simulink model "POWERTRAIN"  (R2026a)
settings: Solver=VariableStepAuto  StopTime=120
InitFcn:
  | Initialize_Project;
undefined symbols (not defined in the file): EV
libraries: SignalEditorBlockLib x1, slpidlib x1
settings Model: Creator=surya  LastModifiedBy=surya

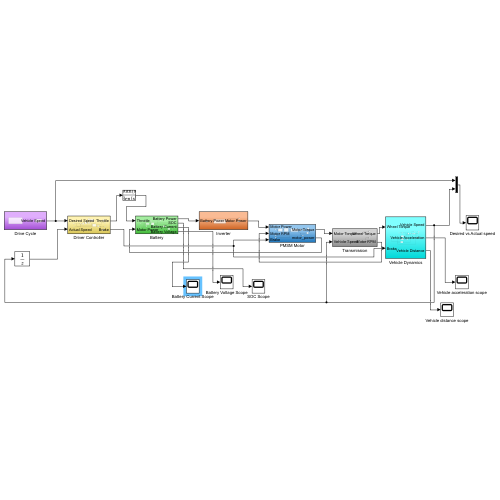
[thumbnail: Simulink's stored preview of the top-level diagram]
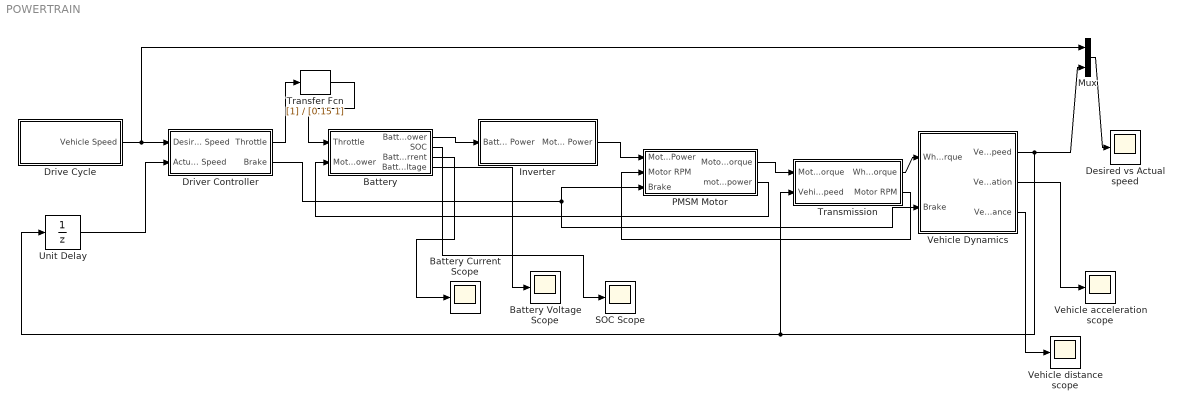
== system POWERTRAIN ==
  Battery : Subsystem
  Battery Current Scope : Scope
      settings: ActiveDisplayYMinimum=-12.119623125546823  ActiveDisplayYMaximum=33.082292003345252  DataLoggingVariableName=ScopeData17
  Battery Voltage Scope : Scope
      settings: ActiveDisplayYMinimum=399.7977387135885  ActiveDisplayYMaximum=400.022473476268  DataLoggingVariableName=ScopeData11
  Desired vs Actual speed : Scope
      settings: ActiveDisplayYMinimum=-2.532730452502121  ActiveDisplayYMaximum=22.794574072519094
  Drive Cycle : Subsystem
  Driver Controller : Subsystem
  Inverter : Subsystem
  Mux : Mux  Inputs=2
  PMSM Motor : Subsystem
  SOC Scope : Scope
      settings: ActiveDisplayYMinimum=99.747173391985541  ActiveDisplayYMaximum=100.02809184533494
  Transfer Fcn : TransferFcn  Denominator=[0.15 1]
  Transmission : Subsystem
  Unit Delay : UnitDelay  SampleTime=-1
  Vehicle Dynamics : Subsystem
  Vehicle acceleration scope : Scope
      settings: ActiveDisplayYMinimum=-1.1905303240766103  ActiveDisplayYMaximum=1.7943093242123052  DataLoggingVariableName=ScopeData6
  Vehicle distance scope : Scope
      settings: ActiveDisplayYMinimum=-118.29137386717078  ActiveDisplayYMaximum=1064.6223648045373  DataLoggingVariableName=ScopeData7
  wires:
  Drive Cycle/1(Vehicle Speed) -> Mux/1, Driver Controller/1(Desired Speed)
  Unit Delay/1 -> Driver Controller/2(Actual Speed)
  Driver Controller/1(Throttle) -> Transfer Fcn/1
  Battery/1(Battery Power) -> Inverter/1(Battery Power)
  Inverter/1(Motor Power) -> PMSM Motor/1(Motor Power)
  PMSM Motor/1(Motor Torque) -> Transmission/1(Motor Torque)
  Transmission/1(Wheel Torque) -> Vehicle Dynamics/1(Wheel Torque)
  Vehicle Dynamics/1(Vehicle Speed) -> Transmission/2(Vehicle Speed), Unit Delay/1, Mux/2
  Battery/2(SOC) -> SOC Scope/1
  Vehicle Dynamics/2(Vehicle Acceleration) -> Vehicle acceleration scope/1
  Vehicle Dynamics/3(Vehicle Distance) -> Vehicle distance scope/1
  Transmission/2(Motor RPM) -> PMSM Motor/2(Motor RPM)
  Transfer Fcn/1 -> Battery/1(Throttle)
  Driver Controller/2(Brake) -> PMSM Motor/3(Brake), Vehicle Dynamics/2(Brake)
  PMSM Motor/2(motor_power) -> Battery/2(Motor Power)
  Battery/3(Battery Current) -> Battery Current Scope/1
  Mux/1 -> Desired vs Actual speed/1
  Battery/4(Battery Voltage) -> Battery Voltage Scope/1

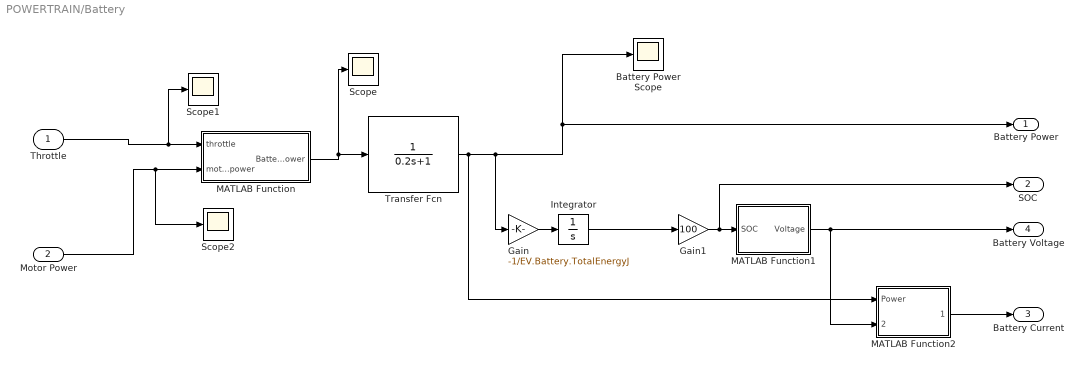
== system POWERTRAIN/Battery ==
  Throttle : Inport
  Motor Power : Inport  Port=2
  Battery Power Scope : Scope
      settings: ActiveDisplayYMinimum=-1  ActiveDisplayYMaximum=1  DataLoggingVariableName=ScopeData2
  Gain : Gain  Gain=-1/EV.Battery.TotalEnergyJ
  Gain1 : Gain  Gain=100
  Integrator : Integrator  InitialCondition=EV.Battery.InitialSOC/100  LimitOutput=on  UpperSaturationLimit=1  LowerSaturationLimit=0
  MATLAB Function : MATLAB Function  TreatAsAtomicUnit=on
  MATLAB Function1 : MATLAB Function  TreatAsAtomicUnit=on
  MATLAB Function2 : MATLAB Function  TreatAsAtomicUnit=on
  Scope : Scope
      settings: ActiveDisplayYMinimum=-1  ActiveDisplayYMaximum=1  DataLoggingVariableName=ScopeData13
  Scope1 : Scope
      settings: ActiveDisplayYMinimum=-1  ActiveDisplayYMaximum=1  DataLoggingVariableName=ScopeData2
  Scope2 : Scope
      settings: ActiveDisplayYMinimum=-1  ActiveDisplayYMaximum=1  DataLoggingVariableName=ScopeData3
  Transfer Fcn : TransferFcn  Denominator=[0.2 1]
  Battery Power : Outport
  SOC : Outport  Port=2
  Battery Current : Outport  Port=3
  Battery Voltage : Outport  Port=4
  wires:
  Throttle/1 -> Scope1/1, MATLAB Function/1(throttle)
  MATLAB Function/1(BatteryPower) -> Scope/1, Transfer Fcn/1
  Transfer Fcn/1 -> MATLAB Function2/1(Power), Gain/1, Battery Power Scope/1, Battery Power/1
  Gain/1 -> Integrator/1
  Integrator/1 -> Gain1/1
  Gain1/1 -> SOC/1, MATLAB Function1/1(SOC)
  Motor Power/1 -> Scope2/1, MATLAB Function/2(motor_power)
  MATLAB Function1/1(Voltage) -> Battery Voltage/1, MATLAB Function2/2(Voltage)
  MATLAB Function2/1(Current) -> Battery Current/1

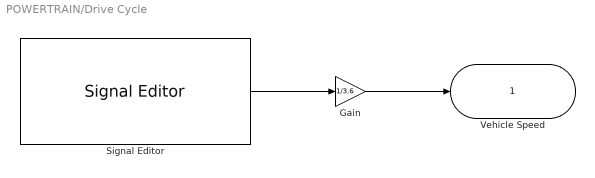
== system POWERTRAIN/Drive Cycle ==
  Gain : Gain  Gain=1/3.6
  Signal Editor : SignalEditorBlockLib/Signal Editor  FileName=C:\Users\surya\OneDrive\Documents\Smart-EV-Powertrain-Simulator\DriveCycles\DriveCycle.mat  ActiveScenario=Scenario  ActiveSignal=Vehicle Speed  IsBus=off  OutputBusObjectStr=Bus: BusObject  SampleTime=0  ZeroCross=off  OutputAfterFinalValue=Setting to zero  Unit=inherit  PreserveSignalName=on  ApplySigPropsToAllScenarios=on  ApplySigPropsToAllSignals=off  SignalPropertySource=Dialog parameters
  Vehicle Speed : Outport
  wires:
  Signal Editor/1 -> Gain/1
  Gain/1 -> Vehicle Speed/1

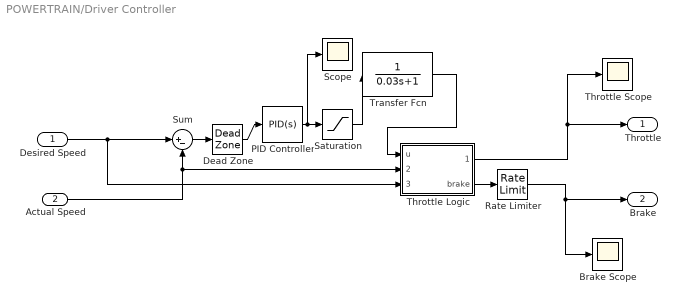
== system POWERTRAIN/Driver Controller ==
  Desired Speed : Inport
  Actual Speed : Inport  Port=2
  Brake Scope : Scope
      settings: ActiveDisplayYMinimum=-1  ActiveDisplayYMaximum=1  DataLoggingVariableName=ScopeData12
  Dead Zone : DeadZone  LowerValue=-0.1  UpperValue=0.1
  PID Controller : slpidlib/PID Controller  Controller=PID  Form=Parallel  TimeDomain=Continuous-time  UseExternalTs=off  SampleTime=-1  IntegratorMethod=Forward Euler  FilterMethod=Forward Euler  ControllerParametersSource=internal  P=0.03  I=0.001  UseKiTs=off  D=0.001  UseExternalDerivativeSource=off  N=20  UseFilter=on  TunerSelectOption=Transfer Function Based (PID Tuner App)  InitialConditionSource=internal  InitialConditionForIntegrator=0  InitialConditionForFilter=0  DifferentiatorICPrevScaledInput=0  ExternalReset=none  TrackingMode=off  Kt=1  LimitOutput=on  SatLimitsSource=internal  UpperSaturationLimit=1  LowerSaturationLimit=-1  LinearizeAsGain=on  AntiWindupMode=back-calculation  Kb=1  LimitIntegrator=off  UpperIntegratorSaturationLimit=inf  LowerIntegratorSaturationLimit=-inf  POutMin=[]  POutMax=[]  IOutMin=[]  IOutMax=[]  DOutMin=[]  DOutMax=[]  NOutMin=[]  NOutMax=[]  SumOutMin=[]  SumOutMax=[]  SaturationOutMin=[]  SaturationOutMax=[]  PParamMin=[]  PParamMax=[]  IParamMin=[]  IParamMax=[]  DParamMin=[]  DParamMax=[]  NParamMin=[]  NParamMax=[]  KbParamMin=[]  KbParamMax=[]  KtParamMin=[]  KtParamMax=[]  KbOutMin=[]  KbOutMax=[]  KtOutMin=[]  KtOutMax=[]  IntegratorOutMin=[]  IntegratorOutMax=[]  FilterOutMin=[]  FilterOutMax=[]  SumI1OutMin=[]  SumI1OutMax=[]  SumI2OutMin=[]  SumI2OutMax=[]  SumI3OutMin=[]  SumI3OutMax=[]  SumI4OutMin=[]  SumI4OutMax=[]  SumDOutMin=[]  SumDOutMax=[]  DifferentiatorOutMin=[]  DifferentiatorOutMax=[]  FilterDiffOutCoefMin=[]  FilterDiffOutCoefMax=[]  ReciprocalOutMin=[]  ReciprocalOutMax=[]  SumDenOutMin=[]  SumDenOutMax=[]  SumNumOutMin=[]  SumNumOutMax=[]  DivideOutMin=[]  DivideOutMax=[]  UdiffTsProdOutMin=[]  UdiffTsProdOutMax=[]  NTsProdOutMin=[]  NTsProdOutMax=[]  UintegralTsProdOutMin=[]  UintegralTsProdOutMax=[]  UngainTsProdOutMin=[]  UngainTsProdOutMax=[]  ClampingZeroOutDataTypeStr=Inherit: Inherit via back propagation  ClampingZeroOutMin=[]  ClampingZeroOutMax=[]  FilterDenConstantOutDataTypeStr=Inherit: Inherit via back propagation  FilterDenConstantOutMin=[]  FilterDenConstantOutMax=[]  PCopyOutDataTypeStr=Inherit: Inherit via back propagation  PCopyOutMin=[]  PCopyOutMax=[]  NCopyOutDataTypeStr=Inherit: Inherit via back propagation  NCopyOutMin=[]  NCopyOutMax=[]  IntegratorContinuousStateAttributes=''  IntegratorStateMustResolveToSignalObject=off  IntegratorRTWStateStorageClass=Auto  FilterContinuousStateAttributes=''  FilterStateMustResolveToSignalObject=off  FilterRTWStateStorageClass=Auto  ParallelPVariant=InternalParameters  IdealPVariant=Disabled  IVariant=InternalParameters  DVariant=InternalParameters  IntegratorVariant=Continuous  SatVariant=Enabled  AWVariant=BackCalculation  PCopyVariant=Disabled  TRVariant=Disabled  FdbkBlocksVariant=Forward  IdealPFdbkVariant=Disabled  SatFdbkVariant=Disabled  DerivativeFilterVariant=ContFilter  NVariant=InternalParameters  NCopyVariant=Disabled  FilterICVariant=InternalICsFilter  IntegratorICVariant=InternalICs  ExternalResetVariant=Disabled  TRSumVariant=Passthrough  SumFdbkVariant=Disabled  SumVariant=Sum_PID  TsampFilterVariant=InternalTs  TsampNgainVariant=Passthrough  TsampIntegralVariant=Disabled_SignalSpec  ExternalSaturationOutDataTypeStr=Inherit: Same as second input  DerivativeSourceVariant=ErrorSignal  PreIntVariant=InternalPreInt
  Rate Limiter : RateLimiter  RisingSlewLimit=0.05  FallingSlewLimit=-0.05  SampleTimeMode=inherited
  Saturation : Saturate  UpperLimit=1  LowerLimit=-1
  Scope : Scope
      settings: ActiveDisplayYMinimum=-1  ActiveDisplayYMaximum=1  DataLoggingVariableName=ScopeData4
  Sum : Sum  Inputs=|+-
  Throttle Logic : MATLAB Function  TreatAsAtomicUnit=on
  Throttle Scope : Scope
      settings: ActiveDisplayYMinimum=-0.028171879428741577  ActiveDisplayYMaximum=0.25354691485867425  DataLoggingVariableName=ScopeData10
  Transfer Fcn : TransferFcn  Denominator=[0.03 1]
  Throttle : Outport  VectorParamsAs1DForOutWhenUnconnected=off
  Brake : Outport  Port=2
  wires:
  Desired Speed/1 -> Throttle Logic/3(desired_speed), Sum/1
  Sum/1 -> Dead Zone/1
  Throttle Logic/1(throttle) -> Throttle/1, Throttle Scope/1
  Actual Speed/1 -> Throttle Logic/2(actual_speed), Sum/2
  Dead Zone/1 -> PID Controller/1
  Throttle Logic/2(brake) -> Rate Limiter/1
  Rate Limiter/1 -> Brake Scope/1, Brake/1
  PID Controller/1 -> Scope/1, Saturation/1
  Saturation/1 -> Transfer Fcn/1
  Transfer Fcn/1 -> Throttle Logic/1(u)

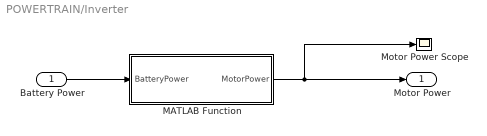
== system POWERTRAIN/Inverter ==
  Battery Power : Inport
  MATLAB Function : MATLAB Function  TreatAsAtomicUnit=on
  Motor Power Scope : Scope
      settings: ActiveDisplayYMinimum=-1  ActiveDisplayYMaximum=1  DataLoggingVariableName=ScopeData9
  Motor Power : Outport
  wires:
  Battery Power/1 -> MATLAB Function/1(BatteryPower)
  MATLAB Function/1(MotorPower) -> Motor Power Scope/1, Motor Power/1

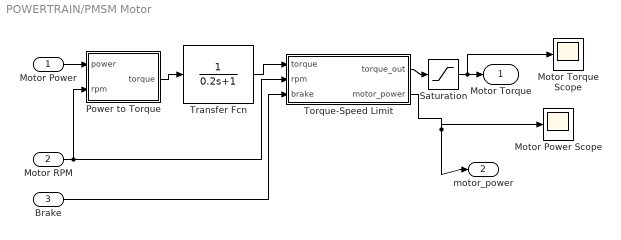
== system POWERTRAIN/PMSM Motor ==
  Motor Power : Inport
  Motor RPM : Inport  Port=2
  Brake : Inport  Port=3
  Motor Power Scope : Scope
      settings: ActiveDisplayYMinimum=-1  ActiveDisplayYMaximum=1  DataLoggingVariableName=ScopeData16
  Motor Torque Scope : Scope
      settings: ActiveDisplayYMinimum=-1  ActiveDisplayYMaximum=1  DataLoggingVariableName=ScopeData4
  Power to Torque : MATLAB Function  TreatAsAtomicUnit=on
  Saturation : Saturate  UpperLimit=EV.Motor.PeakTorque  LowerLimit=-EV.Motor.PeakTorque
  Torque-Speed Limit : MATLAB Function  TreatAsAtomicUnit=on
  Transfer Fcn : TransferFcn  Denominator=[0.2 1]
  Motor Torque : Outport
  motor_power : Outport  Port=2
  wires:
  Motor Power/1 -> Power to Torque/1(power)
  Power to Torque/1(torque) -> Transfer Fcn/1
  Transfer Fcn/1 -> Torque-Speed Limit/1(torque)
  Saturation/1 -> Motor Torque Scope/1, Motor Torque/1
  Torque-Speed Limit/1(torque_out) -> Saturation/1
  Motor RPM/1 -> Power to Torque/2(rpm), Torque-Speed Limit/2(rpm)
  Brake/1 -> Torque-Speed Limit/3(brake)
  Torque-Speed Limit/2(motor_power) -> motor_power/1, Motor Power Scope/1

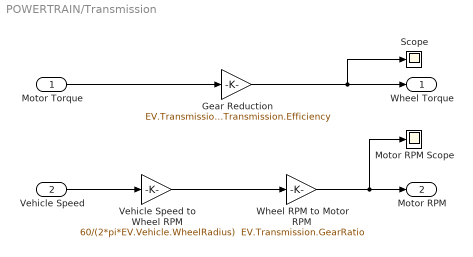
== system POWERTRAIN/Transmission ==
  Motor Torque : Inport
  Vehicle Speed : Inport  Port=2
  Gear Reduction : Gain  Gain=EV.Transmission.GearRatio * EV.Transmission.Efficiency
  Motor RPM Scope : Scope
      settings: ActiveDisplayYMinimum=-1  ActiveDisplayYMaximum=1  DataLoggingVariableName=ScopeData8
  Scope : Scope
      settings: ActiveDisplayYMinimum=-1  ActiveDisplayYMaximum=1  DataLoggingVariableName=ScopeData5
  Vehicle Speed to Wheel RPM : Gain  Gain=60/(2*pi*EV.Vehicle.WheelRadius)
  Wheel RPM to Motor RPM : Gain  Gain=EV.Transmission.GearRatio
  Wheel Torque : Outport
  Motor RPM : Outport  Port=2
  wires:
  Motor Torque/1 -> Gear Reduction/1
  Gear Reduction/1 -> Wheel Torque/1, Scope/1
  Vehicle Speed/1 -> Vehicle Speed to Wheel RPM/1
  Vehicle Speed to Wheel RPM/1 -> Wheel RPM to Motor RPM/1
  Wheel RPM to Motor RPM/1 -> Motor RPM Scope/1, Motor RPM/1

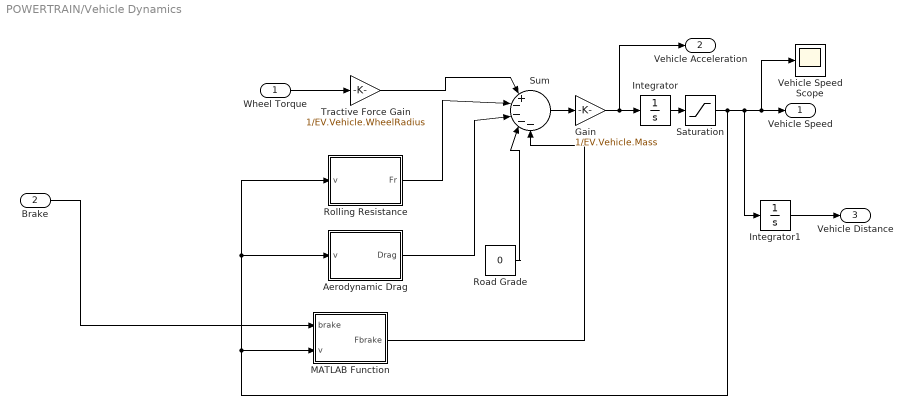
== system POWERTRAIN/Vehicle Dynamics ==
  Wheel Torque : Inport
  Brake : Inport  Port=2
  Aerodynamic Drag : MATLAB Function  TreatAsAtomicUnit=on
  Gain : Gain  Gain=1/EV.Vehicle.Mass
  Integrator : Integrator
  Integrator1 : Integrator
  MATLAB Function : MATLAB Function  TreatAsAtomicUnit=on
  Road Grade : Constant  Value=0
  Rolling Resistance : MATLAB Function  TreatAsAtomicUnit=on
  Saturation : Saturate  UpperLimit=EV.Requirements.TopSpeed  LowerLimit=0
  Sum : Sum  Inputs=|+----
  Tractive Force Gain : Gain  Gain=1/EV.Vehicle.WheelRadius
  Vehicle Speed Scope : Scope
      settings: ActiveDisplayYMinimum=-1  ActiveDisplayYMaximum=1  DataLoggingVariableName=ScopeData3
  Vehicle Speed : Outport
  Vehicle Acceleration : Outport  Port=2
  Vehicle Distance : Outport  Port=3
  wires:
  Wheel Torque/1 -> Tractive Force Gain/1
  Tractive Force Gain/1 -> Sum/1
  Rolling Resistance/1(Fr) -> Sum/2
  Sum/1 -> Gain/1
  Gain/1 -> Integrator/1, Vehicle Acceleration/1
  Integrator/1 -> Saturation/1
  Aerodynamic Drag/1(Drag) -> Sum/3
  Saturation/1 -> Integrator1/1, Vehicle Speed Scope/1, Vehicle Speed/1, Aerodynamic Drag/1(v), Rolling Resistance/1(v), MATLAB Function/2(v)
  Road Grade/1 -> Sum/4
  Integrator1/1 -> Vehicle Distance/1
  Brake/1 -> MATLAB Function/1(brake)
  MATLAB Function/1(Fbrake) -> Sum/5

== matlab function POWERTRAIN/Driver Controller/Throttle Logic ==
  data: u input; throttle output; brake output; actual_speed input; desired_speed input
function [throttle, brake] = fcn(u, actual_speed, desired_speed)

neutral = 0.02;      % Neutral zone around zero

throttle = 0.03;
brake = 0;

% Vehicle stopped
if desired_speed < 0.1 && actual_speed < 0.1

    throttle = 0;
    brake = 0;

    % Accelerate
elseif u > neutral

    throttle = min(u,1);
    brake = 0;

    % Brake
elseif u < -neutral

    throttle = 0;
    brake = min(-u,1);

    % Neutral (no throttle, no brake)
else

    throttle = 0;
    brake = 0;

end

== matlab function POWERTRAIN/PMSM Motor/Power to Torque ==
  data: power input; torque output; rpm input
function torque = fcn(power, rpm)

% Prevent division by zero
rpm_safe = max(abs(rpm),100);

% Convert RPM to rad/s
omega = rpm_safe * 2*pi/60;

% Calculate torque
torque = power / omega;

end

== matlab function POWERTRAIN/Battery/MATLAB Function ==
  data: throttle input; BatteryPower output; motor_power input
function BatteryPower = fcn(throttle,motor_power)

MaxPower = 50000;      % W
DischargeEff = 0.96;
ChargeEff = 0.90;

if motor_power < 0

    % Regenerative charging
    BatteryPower = motor_power * ChargeEff;

else

    RequestedPower = throttle * MaxPower;

    BatteryPower = RequestedPower / DischargeEff;

end

== matlab function POWERTRAIN/Vehicle Dynamics/Aerodynamic Drag ==
  data: v input; Drag output
function Drag = fcn(v)

rho = 1.225;
Cd  = 0.30;
A   = 2.40;

Drag = 0.5 * rho * Cd * A * v * abs(v);

end

== matlab function POWERTRAIN/Vehicle Dynamics/Rolling Resistance ==
  data: v input; Fr output
function Fr = fcn(v)

m = 1650;
g = 9.81;
Cr = 0.01;

if abs(v) < 0.05
    Fr = 0;
else
    Fr = Cr * m * g * sign(v);
end

end

== matlab function POWERTRAIN/PMSM Motor/Torque-Speed Limit ==
  data: torque input; torque_out output; rpm input; brake input; motor_power output
function [torque_out, motor_power] = fcn(torque, rpm, brake)

%% -----------------------------
% Motor Parameters
%% -----------------------------
PeakTorque      = 196.62;      % Nm
RatedTorque     = 167.11;      % Nm

BaseRPM         = 6000;    % Constant torque region
MaxRPM          = 6000;    % Maximum motor speed

MaxRegenTorque  = 120;      % Maximum regenerative torque
MinRegenRPM     = 200;     % Regen fades below this speed

%% -----------------------------
% Forward Driving Torque Limit
%% -----------------------------

if rpm <= BaseRPM

    MaxAllowedTorque = PeakTorque;

elseif rpm < MaxRPM

    % Constant power region
    MaxAllowedTorque = RatedTorque * BaseRPM / rpm;

else

    MaxAllowedTorque = 0;

end

DriveTorque = min(max(torque,0),MaxAllowedTorque);

%% -----------------------------
% Regenerative Braking
%% -----------------------------

if brake > 0

    if rpm >= MinRegenRPM

        RegenFactor = 1;

    else

        % Smoothly reduce regen near zero speed
        RegenFactor = rpm / MinRegenRPM;

    end

    RegenTorque = brake * MaxRegenTorque * RegenFactor;

else

    RegenTorque = 0;

end

%% -----------------------------
% Final Motor Torque
%% -----------------------------

torque_out = DriveTorque - RegenTorque;

%% -----------------------------
% Safety Saturation
%% -----------------------------

if torque_out > PeakTorque
    torque_out = PeakTorque;
end

if torque_out < -MaxRegenTorque
    torque_out = -MaxRegenTorque;
end

%% -----------------------------
% Motor Power
%% -----------------------------

omega = rpm * 2*pi/60;

motor_power = torque_out * omega;

end

== matlab function POWERTRAIN/Battery/MATLAB Function1 ==
  data: SOC input; Voltage output
function Voltage = fcn(SOC)

Vmax = 400;
Vmin = 320;

SOC = max(0,min(100,SOC));

Voltage = Vmin + (Vmax-Vmin)*(SOC/100);

end

== matlab function POWERTRAIN/Battery/MATLAB Function2 ==
  data: Power input; Current output; Voltage input
function Current = fcn(Power,Voltage)

Voltage=max(Voltage,0.1);

Current = Power/Voltage;

end

== matlab function POWERTRAIN/Inverter/MATLAB Function ==
  data: BatteryPower input; MotorPower output
function MotorPower = fcn(BatteryPower)

% Variable inverter efficiency

if abs(BatteryPower) < 1000
    Eff = 0.85;
elseif abs(BatteryPower) < 5000
    Eff = 0.92;
else
    Eff = 0.96;
end

% Battery -> Motor
if BatteryPower >= 0

    MotorPower = BatteryPower * Eff;

    % Motor -> Battery (regenerative braking)
else

    MotorPower = BatteryPower / Eff;

end

end

== matlab function POWERTRAIN/Vehicle Dynamics/MATLAB Function ==
  data: brake input; Fbrake output; v input
function Fbrake = fcn(brake,v)

% Maximum hydraulic braking force
MaxBrakeForce = 10000;   % Newton

if abs(v) < 0.2
    Fbrake = 0;
else
    Fbrake = brake * MaxBrakeForce;
end
